simulink model "lab_01_model"  (R2021a)
settings: Solver=VariableStepAuto  StartTime=0.0  StopTime=0.05  RelTol=1e-3
libraries: spsLinearTransformerLib x2, spsSeriesRLCBranchLib x2, spsACVoltageSourceLib x1, spsCurrentMeasurementLib x1, spsMultimeterLib x1, spsVoltageMeasurementLib x1, spspowerguiLib x1
settings Model: Creator=muham  LastModifiedBy=muham
settings DebuggingCC: UnconnectedInputMsg=none  UnconnectedOutputMsg=none  UnconnectedLineMsg=none

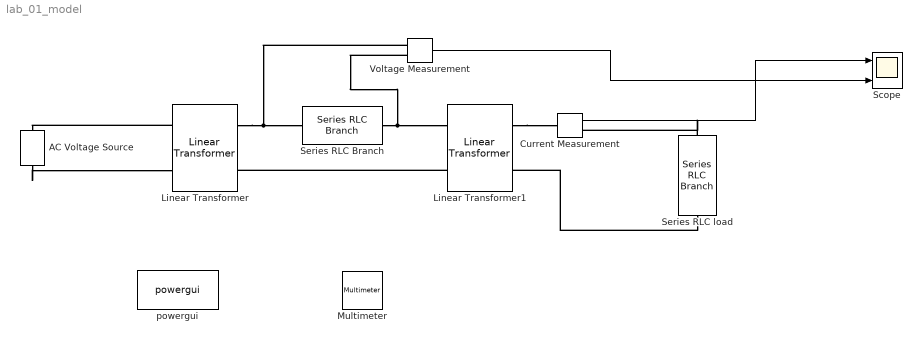
== system lab_01_model ==
  AC Voltage Source : spsACVoltageSourceLib/AC Voltage Source  Amplitude=311.126  Phase=0  Frequency=50  SampleTime=0  Measurements=Voltage  BusType=swing  Pref=10e3  Qref=0  Qmin=-inf  Qmax=+inf
  Current Measurement : spsCurrentMeasurementLib/Current Measurement  PhasorSimulation=off  OutputType=Complex  PSBequivalent=0
  Linear Transformer : spsLinearTransformerLib/Linear Transformer  UNITS=pu  NominalPower=[ 3e3 50 ]  winding1="[ 230  0.002  0.08]"  winding2="[ 433  0.002  0.08 ]"  ThreeWindings=off  winding3=[ 315e3 0.002 0.08 ]  RmLm=[ 500 500 ]  Measurements=All voltages and currents  DataType=off
  Linear Transformer1 : spsLinearTransformerLib/Linear Transformer  UNITS=pu  NominalPower=[ 2e3 50 ]  winding1="[ 440  0.002 0.08 ]"  winding2="[ 120  0.002 0.08]"  ThreeWindings=off  winding3=[ 315e3 0.002 0.08 ]  RmLm=[ 500 500 ]  Measurements=All voltages and currents  DataType=off
  Multimeter : spsMultimeterLib/Multimeter  PhasorSimulation=off  OutputType=Complex  sel=[2 7 8]  L=19  Gain=[1 1 1]  yselected={'Ub: Series RLC load','Usrc: AC Voltage Source','Ib: Series RLC Branch'};  PSBOutputType=1  PSBequivalent=0  AxesSetting=[0,0.1,-100,100]  Display=1  SavedBlockNames=-11
  Scope : Scope  NumInputPorts=2
  Series RLC Branch : spsSeriesRLCBranchLib/Series RLC Branch  LConnTagsString=__new0  RConnTagsString=__new0  BranchType=R  Resistance=3  Inductance=1e-3  SetiL0=off  InitialCurrent=0  Capacitance=1e-6  Setx0=off  InitialVoltage=0  Measurements=Branch voltage and current
  Series RLC load : spsSeriesRLCBranchLib/Series RLC Branch  LConnTagsString=__new0  RConnTagsString=__new0  BranchType=RL  Resistance=0.8  Inductance=0.3/(2*pi*50)  SetiL0=off  InitialCurrent=0  Capacitance=1e-6  Setx0=off  InitialVoltage=0  Measurements=Branch voltage and current
  Voltage Measurement : spsVoltageMeasurementLib/Voltage Measurement  PhasorSimulation=off  OutputType=Complex  PSBequivalent=0
  powergui : spspowerguiLib/powergui  Priority=1  SimulationMode=Continuous  SampleTime=50e-6  frequency=60  Iterations=50  frequencyindice=50  Pbase=100e6  ErrMax=1e-4  UnitsV=kV  UnitsW=MW  buscounter=0  FunctionMessages=off  echomessages=off  EnableUseOfTLC=off  CurrentSourceSwitches=off  DisableSnubberDevices=off  DisableRonSwitches=off  DisableVfSwitches=off  DisplayEquations=off  AutomaticDiscreteSolvers=off  SolverType=Tustin/Backward Euler (TBE)  Interpol=off  ExternalGateDelay=off  methode=off  Ts=100  x0status=steady  SPID=on  SwTol=0  HookPort=off  NonlinearTolerance=1e-4  nMaxIteration=100  ContinueOnMaxIteration=off  RestoreLinks=warning  ResistiveCurrentMeasurement=off  Frange=[0:2:500]  Ylog=off  Xlog=on  ShowGrid=off  save=off  variable=ZData  structure=0  ZoomFFT=off  StartTime=0.0  cycles=1  DisplayStyle=1  fundamental=60  FreqAxis=off  MaxFrequency=1000  frequencyindicesteady=1  RmsSteady=1  display=off
  wires:
  Voltage Measurement/1 -> Scope/2
  Current Measurement/1 -> Scope/1
  connections:
  Linear Transformer/RConn1 -- Voltage Measurement/LConn1 -- Series RLC Branch/LConn1
  Series RLC Branch/RConn1 -- Voltage Measurement/LConn2 -- Linear Transformer1/LConn1
  Linear Transformer1/RConn1 -- Current Measurement/LConn1
  Series RLC load/LConn1 -- Current Measurement/RConn1
  Linear Transformer1/LConn2 -- Linear Transformer/RConn2
  Linear Transformer/LConn1 -- AC Voltage Source/RConn1
  AC Voltage Source/LConn1 -- Linear Transformer/LConn2
  Series RLC load/RConn1 -- Linear Transformer1/RConn2
